simulink model "classd_revb"  (R2024b)
settings: Solver=ode23tb  StartTime=0.0  StopTime=Timespan  MaxStep=classd_maxstep  RelTol=1e-4
InitFcn:
  | p2s_dir = fileparts(get_param(bdroot, 'FileName'));
  | if ~isempty(p2s_dir), addpath(p2s_dir); end
  | clear p2s_dir
  | classd_params;
values from neighbouring files (symbols this model uses):
  Driveshock_freq = 1/(Driveshock_pulse_width*1.25)    (= 72.7272727273)    [classd_params.m]
  Pcd = struct()    [classd_params.m]
  PWMfs = 1/PWMperiod    (= 33333.3333333)    [classd_params.m]
  PWMoffset = PWMperiod/3    (= 1e-05)    [classd_params.m]
  set_current = 450    [classd_params.m]
  shockinterval = 24    [classd_params.m]
  sweep_fEnd = 10000    [classd_params.m]
  sweep_fStart = 4    [classd_params.m]
  tdead = 500e-9    (= 5e-07)    [classd_params.m]
undefined symbols (not defined in the file or in its folder): classd_y0, ipid, vfb
libraries: slpidlib x4
Description:
  | Ideal-switch translation of Class D Rev B.plecs (see README.md)
settings Model: Creator=Jonathan  LastModifiedBy=Jonathan
settings SolverCC: ZeroCrossAlgorithm=Adaptive
settings DebuggingCC: MaxConsecutiveZCsMsg=none

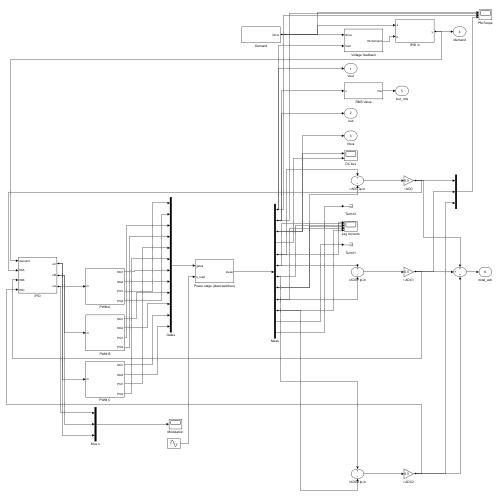
[thumbnail: Simulink's stored preview of the top-level diagram]
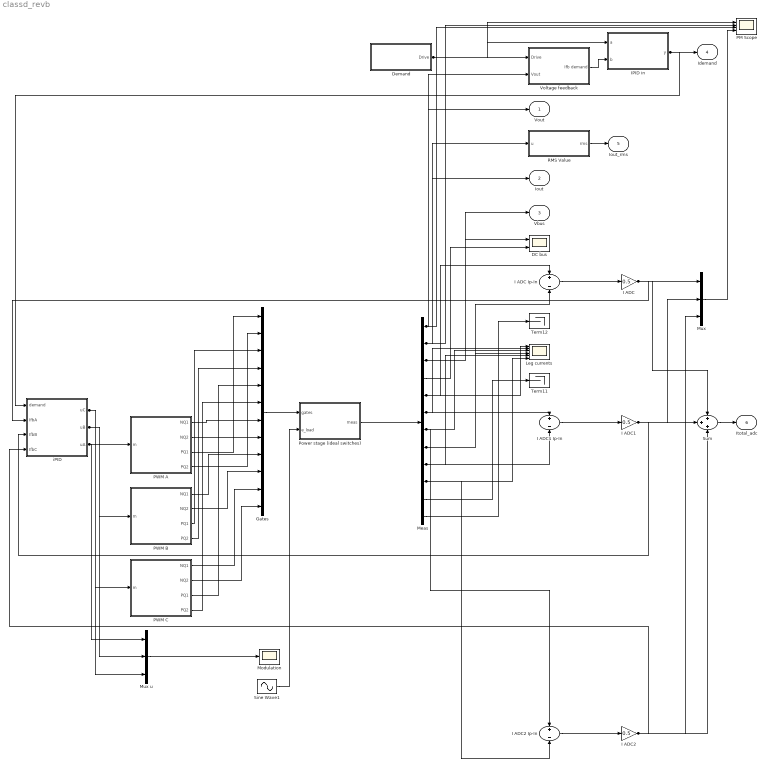
== system classd_revb ==
  DC bus : Scope  NumInputPorts=2
  Demand : Subsystem
  Gates : Mux  Inputs=12
  I ADC : Gain  Gain=0.5
  I ADC Ip-In : Sum  Inputs=+-
  I ADC1 : Gain  Gain=0.5
  I ADC1 Ip-In : Sum  Inputs=+-
  I ADC2 : Gain  Gain=0.5
  I ADC2 Ip-In : Sum  Inputs=+-
  IPID in : Subsystem
  Leg currents : Scope  NumInputPorts=6
  Meas : Demux  Outputs=12
  Modulation : Scope
  Mux : Mux  Inputs=3
  Mux u : Mux  Inputs=3
  PM Scope : Scope  NumInputPorts=4
  PWM A : Subsystem
  PWM B : Subsystem
  PWM C : Subsystem
  Power stage (ideal switches) : Subsystem
  RMS Value : Subsystem
  Sine Wave1 : Sin  Amplitude=10  Frequency=2*pi*20  SampleTime=0
  Sum : Sum  Inputs=+++
  Term11 : Terminator
  Term12 : Terminator
  Voltage feedback : Subsystem
  iPID : Subsystem
  Vout : Outport
  Iout : Outport  Port=2
  Vbus : Outport  Port=3
  Idemand : Outport  Port=4
  Iout_rms : Outport  Port=5
  Itotal_adc : Outport  Port=6
  wires:
  PWM B/4(PQ2) -> Gates/4
  iPID/1(uC) -> PWM C/1(m), Mux u/3
  PWM B/1(NQ1) -> Gates/9
  iPID/2(uB) -> PWM B/1(m), Mux u/2
  iPID/3(uA) -> PWM A/1(m), Mux u/1
  Mux/1 -> PM Scope/4
  PWM A/1(NQ1) -> Gates/7
  PWM A/2(NQ2) -> Gates/8
  PWM A/3(PQ1) -> Gates/1
  PWM A/4(PQ2) -> Gates/2
  PWM B/2(NQ2) -> Gates/10
  PWM B/3(PQ1) -> Gates/3
  Meas/6 -> I ADC1 Ip-In/1, Leg currents/2
  Meas/5 -> Leg currents/1, I ADC Ip-In/1
  PWM C/1(NQ1) -> Gates/11
  PWM C/2(NQ2) -> Gates/12
  Sum/1 -> Itotal_adc/1
  PWM C/4(PQ2) -> Gates/6
  PWM C/3(PQ1) -> Gates/5
  Mux u/1 -> Modulation/1
  Gates/1 -> Power stage (ideal switches)/1(gates)
  Sine Wave1/1 -> Power stage (ideal switches)/2(e_load)
  I ADC1 Ip-In/1 -> I ADC1/1
  Power stage (ideal switches)/1(meas) -> Meas/1
  Demand/1(Drive) -> IPID in/1(a), PM Scope/1, Voltage feedback/1(Drive)
  Meas/2 -> PM Scope/2, RMS Value/1(u), Iout/1
  Meas/1 -> PM Scope/3, Voltage feedback/2(Vout), Vout/1
  Meas/4 -> DC bus/2
  Meas/3 -> DC bus/1, Vbus/1
  Meas/8 -> I ADC Ip-In/2, Leg currents/4
  Meas/7 -> I ADC2 Ip-In/1, Leg currents/3
  Meas/10 -> I ADC2 Ip-In/2, Leg currents/6
  Meas/9 -> I ADC1 Ip-In/2, Leg currents/5
  Meas/12 -> Term12/1
  Meas/11 -> Term11/1
  IPID in/1(y) -> iPID/1(demand), Idemand/1
  Voltage feedback/1(Ifb demand) -> IPID in/2(b)
  RMS Value/1(rms) -> Iout_rms/1
  I ADC Ip-In/1 -> I ADC/1
  I ADC2 Ip-In/1 -> I ADC2/1
  I ADC/1 -> iPID/2(IfbA), Mux/1, Sum/1
  I ADC1/1 -> iPID/3(IfbB), Mux/2, Sum/2
  I ADC2/1 -> iPID/4(IfbC), Sum/3, Mux/3

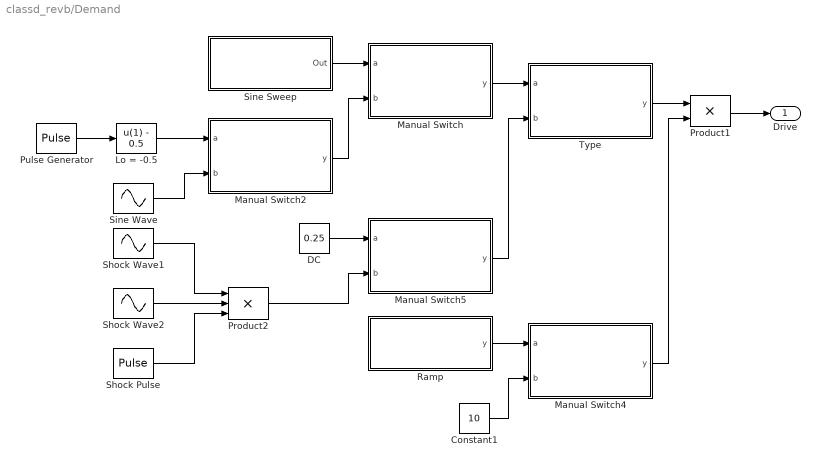
== system classd_revb/Demand ==
  Constant1 : Constant  Value=10
  DC : Constant  Value=0.25
  Lo = -0.5 : Fcn  Expr=u(1) - 0.5
  Manual Switch : Subsystem
  Manual Switch2 : Subsystem
  Manual Switch4 : Subsystem
  Manual Switch5 : Subsystem
  Product1 : Product  Inputs=**
  Product2 : Product  Inputs=***
  Pulse Generator : DiscretePulseGenerator  PulseType=Time based  Period=9/PWMfs  PulseWidth=50  PhaseDelay=0.1
  Ramp : Subsystem
  Shock Pulse : DiscretePulseGenerator  PulseType=Time based  Period=1/(shockinterval*Driveshock_freq/(3*10*2.4))  PulseWidth=100*shockinterval*0.05/2.4
  Shock Wave1 : Sin  Amplitude=set_current  Frequency=2*pi*Driveshock_freq  Phase=-pi  SampleTime=0
  Shock Wave2 : Sin  Amplitude=0.5  Bias=0.5  Frequency=2*pi*Driveshock_freq*2/3  Phase=-pi/2  SampleTime=0
  Sine Sweep : Subsystem
  Sine Wave : Sin  Frequency=2*pi*567.2  SampleTime=0
  Type : Subsystem
  Drive : Outport
  wires:
  Pulse Generator/1 -> Lo = -0.5/1
  Sine Wave/1 -> Manual Switch2/2(b)
  Lo = -0.5/1 -> Manual Switch2/1(a)
  Shock Wave1/1 -> Product2/1
  Sine Sweep/1(Out) -> Manual Switch/1(a)
  Shock Wave2/1 -> Product2/2
  Shock Pulse/1 -> Product2/3
  Manual Switch2/1(y) -> Manual Switch/2(b)
  Product1/1 -> Drive/1
  DC/1 -> Manual Switch5/1(a)
  Product2/1 -> Manual Switch5/2(b)
  Manual Switch/1(y) -> Type/1(a)
  Manual Switch5/1(y) -> Type/2(b)
  Ramp/1(y) -> Manual Switch4/1(a)
  Constant1/1 -> Manual Switch4/2(b)
  Type/1(y) -> Product1/1
  Manual Switch4/1(y) -> Product1/2

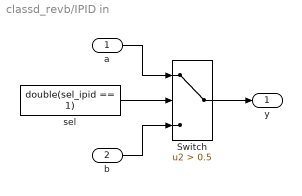
== system classd_revb/IPID in ==
  a : Inport
  b : Inport  Port=2
  Switch : Switch  Criteria=u2 > Threshold  Threshold=0.5  SaturateOnIntegerOverflow=off  InputSameDT=off
  sel : Constant  Value=double(sel_ipid == 1)
  y : Outport
  wires:
  a/1 -> Switch/1
  sel/1 -> Switch/2
  b/1 -> Switch/3
  Switch/1 -> y/1

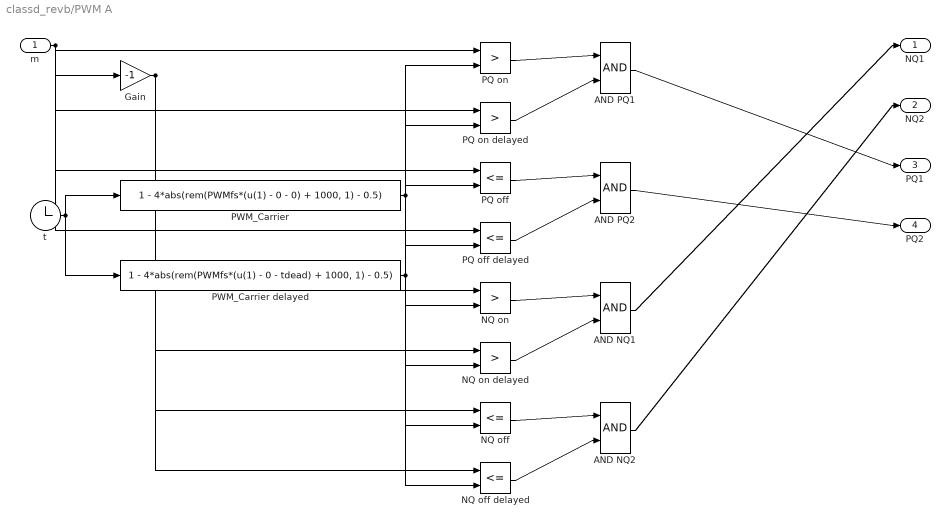
== system classd_revb/PWM A ==
  m : Inport
  AND NQ1 : Logic  AllPortsSameDT=off  OutDataTypeStr=boolean
  AND NQ2 : Logic  AllPortsSameDT=off  OutDataTypeStr=boolean
  AND PQ1 : Logic  AllPortsSameDT=off  OutDataTypeStr=boolean
  AND PQ2 : Logic  AllPortsSameDT=off  OutDataTypeStr=boolean
  Gain : Gain  Gain=-1
  NQ off : RelationalOperator  Operator=<=  OutDataTypeStr=boolean  RndMeth=Simplest  InputSameDT=off
  NQ off delayed : RelationalOperator  Operator=<=  OutDataTypeStr=boolean  RndMeth=Simplest  InputSameDT=off
  NQ on : RelationalOperator  Operator=>  OutDataTypeStr=boolean  RndMeth=Simplest  InputSameDT=off
  NQ on delayed : RelationalOperator  Operator=>  OutDataTypeStr=boolean  RndMeth=Simplest  InputSameDT=off
  PQ off : RelationalOperator  Operator=<=  OutDataTypeStr=boolean  RndMeth=Simplest  InputSameDT=off
  PQ off delayed : RelationalOperator  Operator=<=  OutDataTypeStr=boolean  RndMeth=Simplest  InputSameDT=off
  PQ on : RelationalOperator  Operator=>  OutDataTypeStr=boolean  RndMeth=Simplest  InputSameDT=off
  PQ on delayed : RelationalOperator  Operator=>  OutDataTypeStr=boolean  RndMeth=Simplest  InputSameDT=off
  PWM_Carrier : Fcn  Expr=1 - 4*abs(rem(PWMfs*(u(1) - 0 - 0) + 1000, 1) - 0.5)
  PWM_Carrier delayed : Fcn  Expr=1 - 4*abs(rem(PWMfs*(u(1) - 0 - tdead) + 1000, 1) - 0.5)
  t : Clock
  NQ1 : Outport
  NQ2 : Outport  Port=2
  PQ1 : Outport  Port=3
  PQ2 : Outport  Port=4
  wires:
  t/1 -> PWM_Carrier/1, PWM_Carrier delayed/1
  m/1 -> Gain/1, PQ on/1, PQ on delayed/1, PQ off/1, PQ off delayed/1
  PWM_Carrier/1 -> PQ on/2, PQ off/2, NQ on/2, NQ off/2
  PWM_Carrier delayed/1 -> PQ on delayed/2, PQ off delayed/2, NQ on delayed/2, NQ off delayed/2
  PQ on/1 -> AND PQ1/1
  PQ on delayed/1 -> AND PQ1/2
  PQ off/1 -> AND PQ2/1
  PQ off delayed/1 -> AND PQ2/2
  AND PQ1/1 -> PQ1/1
  AND PQ2/1 -> PQ2/1
  Gain/1 -> NQ on/1, NQ on delayed/1, NQ off/1, NQ off delayed/1
  NQ on/1 -> AND NQ1/1
  NQ on delayed/1 -> AND NQ1/2
  NQ off/1 -> AND NQ2/1
  NQ off delayed/1 -> AND NQ2/2
  AND NQ1/1 -> NQ1/1
  AND NQ2/1 -> NQ2/1

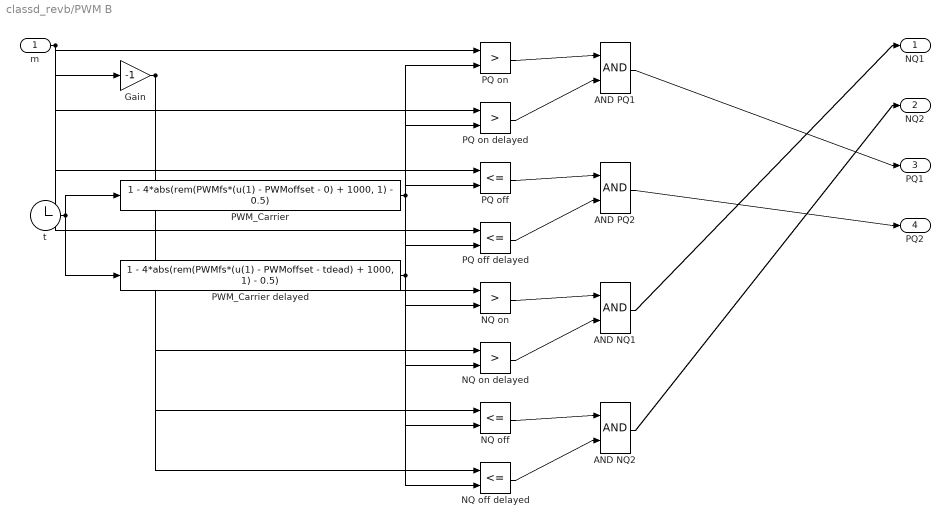
== system classd_revb/PWM B ==
  m : Inport
  AND NQ1 : Logic  AllPortsSameDT=off  OutDataTypeStr=boolean
  AND NQ2 : Logic  AllPortsSameDT=off  OutDataTypeStr=boolean
  AND PQ1 : Logic  AllPortsSameDT=off  OutDataTypeStr=boolean
  AND PQ2 : Logic  AllPortsSameDT=off  OutDataTypeStr=boolean
  Gain : Gain  Gain=-1
  NQ off : RelationalOperator  Operator=<=  OutDataTypeStr=boolean  RndMeth=Simplest  InputSameDT=off
  NQ off delayed : RelationalOperator  Operator=<=  OutDataTypeStr=boolean  RndMeth=Simplest  InputSameDT=off
  NQ on : RelationalOperator  Operator=>  OutDataTypeStr=boolean  RndMeth=Simplest  InputSameDT=off
  NQ on delayed : RelationalOperator  Operator=>  OutDataTypeStr=boolean  RndMeth=Simplest  InputSameDT=off
  PQ off : RelationalOperator  Operator=<=  OutDataTypeStr=boolean  RndMeth=Simplest  InputSameDT=off
  PQ off delayed : RelationalOperator  Operator=<=  OutDataTypeStr=boolean  RndMeth=Simplest  InputSameDT=off
  PQ on : RelationalOperator  Operator=>  OutDataTypeStr=boolean  RndMeth=Simplest  InputSameDT=off
  PQ on delayed : RelationalOperator  Operator=>  OutDataTypeStr=boolean  RndMeth=Simplest  InputSameDT=off
  PWM_Carrier : Fcn  Expr=1 - 4*abs(rem(PWMfs*(u(1) - PWMoffset - 0) + 1000, 1) - 0.5)
  PWM_Carrier delayed : Fcn  Expr=1 - 4*abs(rem(PWMfs*(u(1) - PWMoffset - tdead) + 1000, 1) - 0.5)
  t : Clock
  NQ1 : Outport
  NQ2 : Outport  Port=2
  PQ1 : Outport  Port=3
  PQ2 : Outport  Port=4
  wires:
  t/1 -> PWM_Carrier/1, PWM_Carrier delayed/1
  m/1 -> Gain/1, PQ on/1, PQ on delayed/1, PQ off/1, PQ off delayed/1
  PWM_Carrier/1 -> PQ on/2, PQ off/2, NQ on/2, NQ off/2
  PWM_Carrier delayed/1 -> PQ on delayed/2, PQ off delayed/2, NQ on delayed/2, NQ off delayed/2
  PQ on/1 -> AND PQ1/1
  PQ on delayed/1 -> AND PQ1/2
  PQ off/1 -> AND PQ2/1
  PQ off delayed/1 -> AND PQ2/2
  AND PQ1/1 -> PQ1/1
  AND PQ2/1 -> PQ2/1
  Gain/1 -> NQ on/1, NQ on delayed/1, NQ off/1, NQ off delayed/1
  NQ on/1 -> AND NQ1/1
  NQ on delayed/1 -> AND NQ1/2
  NQ off/1 -> AND NQ2/1
  NQ off delayed/1 -> AND NQ2/2
  AND NQ1/1 -> NQ1/1
  AND NQ2/1 -> NQ2/1

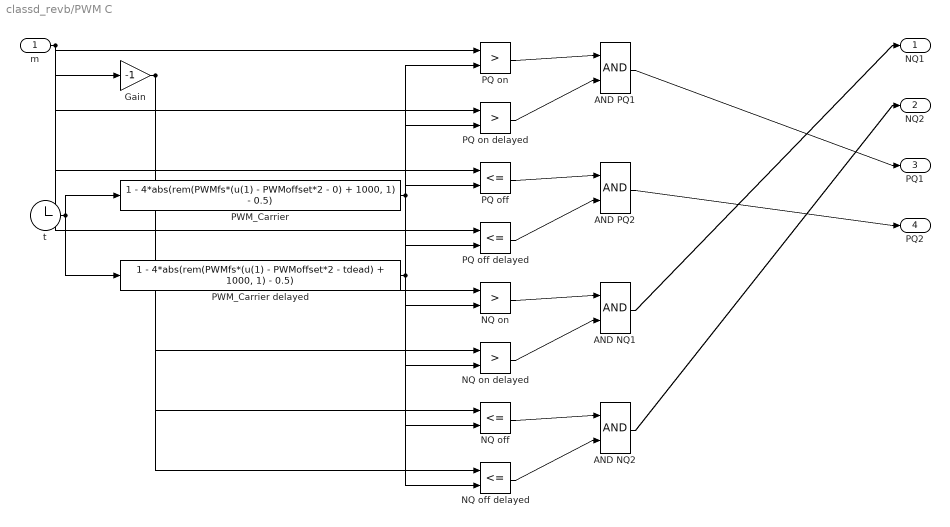
== system classd_revb/PWM C ==
  m : Inport
  AND NQ1 : Logic  AllPortsSameDT=off  OutDataTypeStr=boolean
  AND NQ2 : Logic  AllPortsSameDT=off  OutDataTypeStr=boolean
  AND PQ1 : Logic  AllPortsSameDT=off  OutDataTypeStr=boolean
  AND PQ2 : Logic  AllPortsSameDT=off  OutDataTypeStr=boolean
  Gain : Gain  Gain=-1
  NQ off : RelationalOperator  Operator=<=  OutDataTypeStr=boolean  RndMeth=Simplest  InputSameDT=off
  NQ off delayed : RelationalOperator  Operator=<=  OutDataTypeStr=boolean  RndMeth=Simplest  InputSameDT=off
  NQ on : RelationalOperator  Operator=>  OutDataTypeStr=boolean  RndMeth=Simplest  InputSameDT=off
  NQ on delayed : RelationalOperator  Operator=>  OutDataTypeStr=boolean  RndMeth=Simplest  InputSameDT=off
  PQ off : RelationalOperator  Operator=<=  OutDataTypeStr=boolean  RndMeth=Simplest  InputSameDT=off
  PQ off delayed : RelationalOperator  Operator=<=  OutDataTypeStr=boolean  RndMeth=Simplest  InputSameDT=off
  PQ on : RelationalOperator  Operator=>  OutDataTypeStr=boolean  RndMeth=Simplest  InputSameDT=off
  PQ on delayed : RelationalOperator  Operator=>  OutDataTypeStr=boolean  RndMeth=Simplest  InputSameDT=off
  PWM_Carrier : Fcn  Expr=1 - 4*abs(rem(PWMfs*(u(1) - PWMoffset*2 - 0) + 1000, 1) - 0.5)
  PWM_Carrier delayed : Fcn  Expr=1 - 4*abs(rem(PWMfs*(u(1) - PWMoffset*2 - tdead) + 1000, 1) - 0.5)
  t : Clock
  NQ1 : Outport
  NQ2 : Outport  Port=2
  PQ1 : Outport  Port=3
  PQ2 : Outport  Port=4
  wires:
  t/1 -> PWM_Carrier/1, PWM_Carrier delayed/1
  m/1 -> Gain/1, PQ on/1, PQ on delayed/1, PQ off/1, PQ off delayed/1
  PWM_Carrier/1 -> PQ on/2, PQ off/2, NQ on/2, NQ off/2
  PWM_Carrier delayed/1 -> PQ on delayed/2, PQ off delayed/2, NQ on delayed/2, NQ off delayed/2
  PQ on/1 -> AND PQ1/1
  PQ on delayed/1 -> AND PQ1/2
  PQ off/1 -> AND PQ2/1
  PQ off delayed/1 -> AND PQ2/2
  AND PQ1/1 -> PQ1/1
  AND PQ2/1 -> PQ2/1
  Gain/1 -> NQ on/1, NQ on delayed/1, NQ off/1, NQ off delayed/1
  NQ on/1 -> AND NQ1/1
  NQ on delayed/1 -> AND NQ1/2
  NQ off/1 -> AND NQ2/1
  NQ off delayed/1 -> AND NQ2/2
  AND NQ1/1 -> NQ1/1
  AND NQ2/1 -> NQ2/1

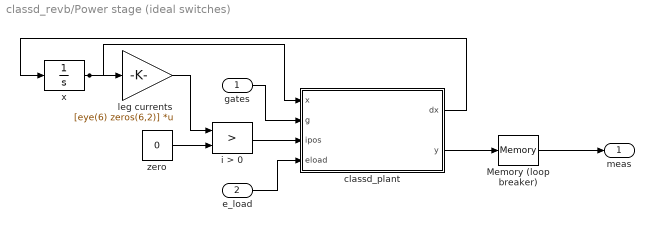
== system classd_revb/Power stage (ideal switches) ==
  gates : Inport
  e_load : Inport  Port=2
  Memory (loop breaker) : Memory  InitialCondition=classd_y0
  classd_plant : MATLAB Function  TreatAsAtomicUnit=on
  i > 0 : RelationalOperator  Operator=>  OutDataTypeStr=boolean  RndMeth=Simplest  InputSameDT=off
  leg currents : Gain  Gain=[eye(6) zeros(6,2)]  Multiplication=Matrix(K*u)
  x : Integrator  InitialCondition=Pcd.x0
  zero : Constant  Value=0
  meas : Outport
  wires:
  classd_plant/2(y) -> Memory (loop breaker)/1
  x/1 -> classd_plant/1(x), leg currents/1
  leg currents/1 -> i > 0/1
  classd_plant/1(dx) -> x/1
  zero/1 -> i > 0/2
  e_load/1 -> classd_plant/4(eload)
  gates/1 -> classd_plant/2(g)
  i > 0/1 -> classd_plant/3(ipos)
  Memory (loop breaker)/1 -> meas/1

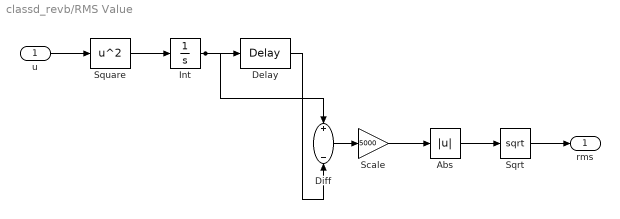
== system classd_revb/RMS Value ==
  u : Inport
  Abs : Abs  SaturateOnIntegerOverflow=off
  Delay : TransportDelay  DelayTime=1/(5000)  BufferSize=131072
  Diff : Sum  Inputs=+-
  Int : Integrator
  Scale : Gain  Gain=5000
  Sqrt : Sqrt
  Square : Math  Operator=square
  rms : Outport
  wires:
  Diff/1 -> Scale/1
  u/1 -> Square/1
  Square/1 -> Int/1
  Delay/1 -> Diff/2
  Int/1 -> Diff/1, Delay/1
  Scale/1 -> Abs/1
  Abs/1 -> Sqrt/1
  Sqrt/1 -> rms/1

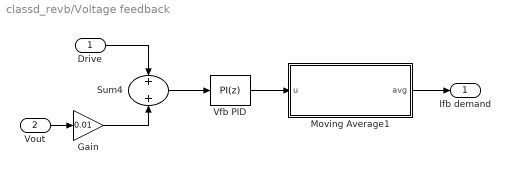
== system classd_revb/Voltage feedback ==
  Drive : Inport
  Vout : Inport  Port=2
  Gain : Gain  Gain=0.01
  Moving Average1 : Subsystem
  Sum4 : Sum
  Vfb PID : slpidlib/PID Controller  Controller=PI  Form=Parallel  TimeDomain=Discrete-time  UseExternalTs=off  SampleTime=vfb.Ts  IntegratorMethod=Forward Euler  FilterMethod=Forward Euler  ControllerParametersSource=internal  P=vfb.kp  I=vfb.ki  UseKiTs=off  D=0  UseExternalDerivativeSource=off  N=100  UseFilter=on  TunerSelectOption=Transfer Function Based (PID Tuner App)  InitialConditionSource=internal  InitialConditionForIntegrator=0  InitialConditionForFilter=0  DifferentiatorICPrevScaledInput=0  ExternalReset=none  TrackingMode=off  Kt=1  LimitOutput=on  SatLimitsSource=internal  UpperSaturationLimit=vfb.up  LowerSaturationLimit=vfb.lo  LinearizeAsGain=off  AntiWindupMode=clamping  Kb=1  LimitIntegrator=off  UpperIntegratorSaturationLimit=inf  LowerIntegratorSaturationLimit=-inf  POutMin=[]  POutMax=[]  IOutMin=[]  IOutMax=[]  DOutMin=[]  DOutMax=[]  NOutMin=[]  NOutMax=[]  SumOutMin=[]  SumOutMax=[]  SaturationOutMin=[]  SaturationOutMax=[]  PParamMin=[]  PParamMax=[]  IParamMin=[]  IParamMax=[]  DParamMin=[]  DParamMax=[]  NParamMin=[]  NParamMax=[]  KbParamMin=[]  KbParamMax=[]  KtParamMin=[]  KtParamMax=[]  KbOutMin=[]  KbOutMax=[]  KtOutMin=[]  KtOutMax=[]  IntegratorOutMin=[]  IntegratorOutMax=[]  FilterOutMin=[]  FilterOutMax=[]  SumI1OutMin=[]  SumI1OutMax=[]  SumI2OutMin=[]  SumI2OutMax=[]  SumI3OutMin=[]  SumI3OutMax=[]  SumI4OutMin=[]  SumI4OutMax=[]  SumDOutMin=[]  SumDOutMax=[]  DifferentiatorOutMin=[]  DifferentiatorOutMax=[]  FilterDiffOutCoefMin=[]  FilterDiffOutCoefMax=[]  ReciprocalOutMin=[]  ReciprocalOutMax=[]  SumDenOutMin=[]  SumDenOutMax=[]  SumNumOutMin=[]  SumNumOutMax=[]  DivideOutMin=[]  DivideOutMax=[]  UdiffTsProdOutMin=[]  UdiffTsProdOutMax=[]  NTsProdOutMin=[]  NTsProdOutMax=[]  UintegralTsProdOutMin=[]  UintegralTsProdOutMax=[]  UngainTsProdOutMin=[]  UngainTsProdOutMax=[]  ClampingZeroOutDataTypeStr=Inherit: Inherit via back propagation  ClampingZeroOutMin=[]  ClampingZeroOutMax=[]  FilterDenConstantOutDataTypeStr=Inherit: Inherit via back propagation  FilterDenConstantOutMin=[]  FilterDenConstantOutMax=[]  PCopyOutDataTypeStr=Inherit: Inherit via back propagation  PCopyOutMin=[]  PCopyOutMax=[]  NCopyOutDataTypeStr=Inherit: Inherit via back propagation  NCopyOutMin=[]  NCopyOutMax=[]  IntegratorContinuousStateAttributes=''  IntegratorStateMustResolveToSignalObject=off  IntegratorRTWStateStorageClass=Auto  FilterContinuousStateAttributes=''  FilterStateMustResolveToSignalObject=off  FilterRTWStateStorageClass=Auto  ParallelPVariant=InternalParameters  IdealPVariant=Disabled  IVariant=InternalParameters  DVariant=Disabled  IntegratorVariant=Discrete  SatVariant=Enabled  AWVariant=DiscClampingParallel  PCopyVariant=Disabled  TRVariant=Disabled  FdbkBlocksVariant=Forward  IdealPFdbkVariant=Disabled  SatFdbkVariant=Disabled  DerivativeFilterVariant=Disabled  NVariant=Disabled  NCopyVariant=Disabled_SignalSpec  FilterICVariant=Disabled  IntegratorICVariant=InternalICs  ExternalResetVariant=Disabled  TRSumVariant=Passthrough  SumFdbkVariant=Disabled  SumVariant=Sum_PI  TsampFilterVariant=InternalTs  TsampNgainVariant=Passthrough  TsampIntegralVariant=Disabled_SignalSpec  ExternalSaturationOutDataTypeStr=Inherit: Same as second input  DerivativeSourceVariant=Disabled  PreIntVariant=InternalPreInt
      settings: LibrarySourceBlock=simulink/Discrete/Discrete PID Controller
  Ifb demand : Outport
  wires:
  Vout/1 -> Gain/1
  Moving Average1/1(avg) -> Ifb demand/1
  Drive/1 -> Sum4/1
  Gain/1 -> Sum4/2
  Sum4/1 -> Vfb PID/1
  Vfb PID/1 -> Moving Average1/1(u)

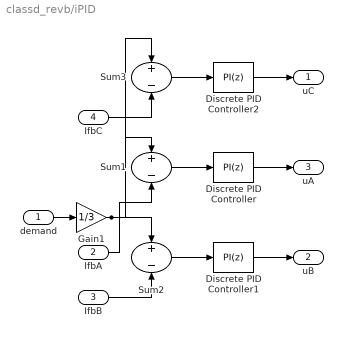
== system classd_revb/iPID ==
  demand : Inport
  IfbA : Inport  Port=2
  IfbB : Inport  Port=3
  IfbC : Inport  Port=4
  Discrete PID Controller : slpidlib/PID Controller  Controller=PI  Form=Parallel  TimeDomain=Discrete-time  UseExternalTs=off  SampleTime=ipid.Ts  IntegratorMethod=Forward Euler  FilterMethod=Forward Euler  ControllerParametersSource=internal  P=ipid.kp  I=ipid.ki  UseKiTs=off  D=0  UseExternalDerivativeSource=off  N=100  UseFilter=on  TunerSelectOption=Transfer Function Based (PID Tuner App)  InitialConditionSource=internal  InitialConditionForIntegrator=0  InitialConditionForFilter=0  DifferentiatorICPrevScaledInput=0  ExternalReset=none  TrackingMode=off  Kt=1  LimitOutput=on  SatLimitsSource=internal  UpperSaturationLimit=ipid.up  LowerSaturationLimit=ipid.lo  LinearizeAsGain=off  AntiWindupMode=back-calculation  Kb=ipid.kbc  LimitIntegrator=off  UpperIntegratorSaturationLimit=inf  LowerIntegratorSaturationLimit=-inf  POutMin=[]  POutMax=[]  IOutMin=[]  IOutMax=[]  DOutMin=[]  DOutMax=[]  NOutMin=[]  NOutMax=[]  SumOutMin=[]  SumOutMax=[]  SaturationOutMin=[]  SaturationOutMax=[]  PParamMin=[]  PParamMax=[]  IParamMin=[]  IParamMax=[]  DParamMin=[]  DParamMax=[]  NParamMin=[]  NParamMax=[]  KbParamMin=[]  KbParamMax=[]  KtParamMin=[]  KtParamMax=[]  KbOutMin=[]  KbOutMax=[]  KtOutMin=[]  KtOutMax=[]  IntegratorOutMin=[]  IntegratorOutMax=[]  FilterOutMin=[]  FilterOutMax=[]  SumI1OutMin=[]  SumI1OutMax=[]  SumI2OutMin=[]  SumI2OutMax=[]  SumI3OutMin=[]  SumI3OutMax=[]  SumI4OutMin=[]  SumI4OutMax=[]  SumDOutMin=[]  SumDOutMax=[]  DifferentiatorOutMin=[]  DifferentiatorOutMax=[]  FilterDiffOutCoefMin=[]  FilterDiffOutCoefMax=[]  ReciprocalOutMin=[]  ReciprocalOutMax=[]  SumDenOutMin=[]  SumDenOutMax=[]  SumNumOutMin=[]  SumNumOutMax=[]  DivideOutMin=[]  DivideOutMax=[]  UdiffTsProdOutMin=[]  UdiffTsProdOutMax=[]  NTsProdOutMin=[]  NTsProdOutMax=[]  UintegralTsProdOutMin=[]  UintegralTsProdOutMax=[]  UngainTsProdOutMin=[]  UngainTsProdOutMax=[]  ClampingZeroOutDataTypeStr=Inherit: Inherit via back propagation  ClampingZeroOutMin=[]  ClampingZeroOutMax=[]  FilterDenConstantOutDataTypeStr=Inherit: Inherit via back propagation  FilterDenConstantOutMin=[]  FilterDenConstantOutMax=[]  PCopyOutDataTypeStr=Inherit: Inherit via back propagation  PCopyOutMin=[]  PCopyOutMax=[]  NCopyOutDataTypeStr=Inherit: Inherit via back propagation  NCopyOutMin=[]  NCopyOutMax=[]  IntegratorContinuousStateAttributes=''  IntegratorStateMustResolveToSignalObject=off  IntegratorRTWStateStorageClass=Auto  FilterContinuousStateAttributes=''  FilterStateMustResolveToSignalObject=off  FilterRTWStateStorageClass=Auto  ParallelPVariant=InternalParameters  IdealPVariant=Disabled  IVariant=InternalParameters  DVariant=Disabled  IntegratorVariant=Discrete  SatVariant=Enabled  AWVariant=BackCalculation  PCopyVariant=Disabled  TRVariant=Disabled  FdbkBlocksVariant=Forward  IdealPFdbkVariant=Disabled  SatFdbkVariant=Disabled  DerivativeFilterVariant=Disabled  NVariant=Disabled  NCopyVariant=Disabled_SignalSpec  FilterICVariant=Disabled  IntegratorICVariant=InternalICs  ExternalResetVariant=Disabled  TRSumVariant=Passthrough  SumFdbkVariant=Disabled  SumVariant=Sum_PI  TsampFilterVariant=InternalTs  TsampNgainVariant=Passthrough  TsampIntegralVariant=Disabled_SignalSpec  ExternalSaturationOutDataTypeStr=Inherit: Same as second input  DerivativeSourceVariant=Disabled  PreIntVariant=InternalPreInt
      settings: LibrarySourceBlock=simulink/Discrete/Discrete PID Controller
  Discrete PID Controller1 : slpidlib/PID Controller  Controller=PI  Form=Parallel  TimeDomain=Discrete-time  UseExternalTs=off  SampleTime=ipid.Ts  IntegratorMethod=Forward Euler  FilterMethod=Forward Euler  ControllerParametersSource=internal  P=ipid.kp  I=ipid.ki  UseKiTs=off  D=0  UseExternalDerivativeSource=off  N=100  UseFilter=on  TunerSelectOption=Transfer Function Based (PID Tuner App)  InitialConditionSource=internal  InitialConditionForIntegrator=0  InitialConditionForFilter=0  DifferentiatorICPrevScaledInput=0  ExternalReset=none  TrackingMode=off  Kt=1  LimitOutput=on  SatLimitsSource=internal  UpperSaturationLimit=ipid.up  LowerSaturationLimit=ipid.lo  LinearizeAsGain=off  AntiWindupMode=back-calculation  Kb=ipid.kbc  LimitIntegrator=off  UpperIntegratorSaturationLimit=inf  LowerIntegratorSaturationLimit=-inf  POutMin=[]  POutMax=[]  IOutMin=[]  IOutMax=[]  DOutMin=[]  DOutMax=[]  NOutMin=[]  NOutMax=[]  SumOutMin=[]  SumOutMax=[]  SaturationOutMin=[]  SaturationOutMax=[]  PParamMin=[]  PParamMax=[]  IParamMin=[]  IParamMax=[]  DParamMin=[]  DParamMax=[]  NParamMin=[]  NParamMax=[]  KbParamMin=[]  KbParamMax=[]  KtParamMin=[]  KtParamMax=[]  KbOutMin=[]  KbOutMax=[]  KtOutMin=[]  KtOutMax=[]  IntegratorOutMin=[]  IntegratorOutMax=[]  FilterOutMin=[]  FilterOutMax=[]  SumI1OutMin=[]  SumI1OutMax=[]  SumI2OutMin=[]  SumI2OutMax=[]  SumI3OutMin=[]  SumI3OutMax=[]  SumI4OutMin=[]  SumI4OutMax=[]  SumDOutMin=[]  SumDOutMax=[]  DifferentiatorOutMin=[]  DifferentiatorOutMax=[]  FilterDiffOutCoefMin=[]  FilterDiffOutCoefMax=[]  ReciprocalOutMin=[]  ReciprocalOutMax=[]  SumDenOutMin=[]  SumDenOutMax=[]  SumNumOutMin=[]  SumNumOutMax=[]  DivideOutMin=[]  DivideOutMax=[]  UdiffTsProdOutMin=[]  UdiffTsProdOutMax=[]  NTsProdOutMin=[]  NTsProdOutMax=[]  UintegralTsProdOutMin=[]  UintegralTsProdOutMax=[]  UngainTsProdOutMin=[]  UngainTsProdOutMax=[]  ClampingZeroOutDataTypeStr=Inherit: Inherit via back propagation  ClampingZeroOutMin=[]  ClampingZeroOutMax=[]  FilterDenConstantOutDataTypeStr=Inherit: Inherit via back propagation  FilterDenConstantOutMin=[]  FilterDenConstantOutMax=[]  PCopyOutDataTypeStr=Inherit: Inherit via back propagation  PCopyOutMin=[]  PCopyOutMax=[]  NCopyOutDataTypeStr=Inherit: Inherit via back propagation  NCopyOutMin=[]  NCopyOutMax=[]  IntegratorContinuousStateAttributes=''  IntegratorStateMustResolveToSignalObject=off  IntegratorRTWStateStorageClass=Auto  FilterContinuousStateAttributes=''  FilterStateMustResolveToSignalObject=off  FilterRTWStateStorageClass=Auto  ParallelPVariant=InternalParameters  IdealPVariant=Disabled  IVariant=InternalParameters  DVariant=Disabled  IntegratorVariant=Discrete  SatVariant=Enabled  AWVariant=BackCalculation  PCopyVariant=Disabled  TRVariant=Disabled  FdbkBlocksVariant=Forward  IdealPFdbkVariant=Disabled  SatFdbkVariant=Disabled  DerivativeFilterVariant=Disabled  NVariant=Disabled  NCopyVariant=Disabled_SignalSpec  FilterICVariant=Disabled  IntegratorICVariant=InternalICs  ExternalResetVariant=Disabled  TRSumVariant=Passthrough  SumFdbkVariant=Disabled  SumVariant=Sum_PI  TsampFilterVariant=InternalTs  TsampNgainVariant=Passthrough  TsampIntegralVariant=Disabled_SignalSpec  ExternalSaturationOutDataTypeStr=Inherit: Same as second input  DerivativeSourceVariant=Disabled  PreIntVariant=InternalPreInt
      settings: LibrarySourceBlock=simulink/Discrete/Discrete PID Controller
  Discrete PID Controller2 : slpidlib/PID Controller  Controller=PI  Form=Parallel  TimeDomain=Discrete-time  UseExternalTs=off  SampleTime=ipid.Ts  IntegratorMethod=Forward Euler  FilterMethod=Forward Euler  ControllerParametersSource=internal  P=ipid.kp  I=ipid.ki  UseKiTs=off  D=0  UseExternalDerivativeSource=off  N=100  UseFilter=on  TunerSelectOption=Transfer Function Based (PID Tuner App)  InitialConditionSource=internal  InitialConditionForIntegrator=0  InitialConditionForFilter=0  DifferentiatorICPrevScaledInput=0  ExternalReset=none  TrackingMode=off  Kt=1  LimitOutput=on  SatLimitsSource=internal  UpperSaturationLimit=ipid.up  LowerSaturationLimit=ipid.lo  LinearizeAsGain=off  AntiWindupMode=back-calculation  Kb=ipid.kbc  LimitIntegrator=off  UpperIntegratorSaturationLimit=inf  LowerIntegratorSaturationLimit=-inf  POutMin=[]  POutMax=[]  IOutMin=[]  IOutMax=[]  DOutMin=[]  DOutMax=[]  NOutMin=[]  NOutMax=[]  SumOutMin=[]  SumOutMax=[]  SaturationOutMin=[]  SaturationOutMax=[]  PParamMin=[]  PParamMax=[]  IParamMin=[]  IParamMax=[]  DParamMin=[]  DParamMax=[]  NParamMin=[]  NParamMax=[]  KbParamMin=[]  KbParamMax=[]  KtParamMin=[]  KtParamMax=[]  KbOutMin=[]  KbOutMax=[]  KtOutMin=[]  KtOutMax=[]  IntegratorOutMin=[]  IntegratorOutMax=[]  FilterOutMin=[]  FilterOutMax=[]  SumI1OutMin=[]  SumI1OutMax=[]  SumI2OutMin=[]  SumI2OutMax=[]  SumI3OutMin=[]  SumI3OutMax=[]  SumI4OutMin=[]  SumI4OutMax=[]  SumDOutMin=[]  SumDOutMax=[]  DifferentiatorOutMin=[]  DifferentiatorOutMax=[]  FilterDiffOutCoefMin=[]  FilterDiffOutCoefMax=[]  ReciprocalOutMin=[]  ReciprocalOutMax=[]  SumDenOutMin=[]  SumDenOutMax=[]  SumNumOutMin=[]  SumNumOutMax=[]  DivideOutMin=[]  DivideOutMax=[]  UdiffTsProdOutMin=[]  UdiffTsProdOutMax=[]  NTsProdOutMin=[]  NTsProdOutMax=[]  UintegralTsProdOutMin=[]  UintegralTsProdOutMax=[]  UngainTsProdOutMin=[]  UngainTsProdOutMax=[]  ClampingZeroOutDataTypeStr=Inherit: Inherit via back propagation  ClampingZeroOutMin=[]  ClampingZeroOutMax=[]  FilterDenConstantOutDataTypeStr=Inherit: Inherit via back propagation  FilterDenConstantOutMin=[]  FilterDenConstantOutMax=[]  PCopyOutDataTypeStr=Inherit: Inherit via back propagation  PCopyOutMin=[]  PCopyOutMax=[]  NCopyOutDataTypeStr=Inherit: Inherit via back propagation  NCopyOutMin=[]  NCopyOutMax=[]  IntegratorContinuousStateAttributes=''  IntegratorStateMustResolveToSignalObject=off  IntegratorRTWStateStorageClass=Auto  FilterContinuousStateAttributes=''  FilterStateMustResolveToSignalObject=off  FilterRTWStateStorageClass=Auto  ParallelPVariant=InternalParameters  IdealPVariant=Disabled  IVariant=InternalParameters  DVariant=Disabled  IntegratorVariant=Discrete  SatVariant=Enabled  AWVariant=BackCalculation  PCopyVariant=Disabled  TRVariant=Disabled  FdbkBlocksVariant=Forward  IdealPFdbkVariant=Disabled  SatFdbkVariant=Disabled  DerivativeFilterVariant=Disabled  NVariant=Disabled  NCopyVariant=Disabled_SignalSpec  FilterICVariant=Disabled  IntegratorICVariant=InternalICs  ExternalResetVariant=Disabled  TRSumVariant=Passthrough  SumFdbkVariant=Disabled  SumVariant=Sum_PI  TsampFilterVariant=InternalTs  TsampNgainVariant=Passthrough  TsampIntegralVariant=Disabled_SignalSpec  ExternalSaturationOutDataTypeStr=Inherit: Same as second input  DerivativeSourceVariant=Disabled  PreIntVariant=InternalPreInt
      settings: LibrarySourceBlock=simulink/Discrete/Discrete PID Controller
  Gain1 : Gain  Gain=1/3
  Sum1 : Sum  Inputs=+-
  Sum2 : Sum  Inputs=+-
  Sum3 : Sum  Inputs=+-
  uC : Outport
  uB : Outport  Port=2
  uA : Outport  Port=3
  wires:
  demand/1 -> Gain1/1
  IfbC/1 -> Sum3/2
  IfbB/1 -> Sum2/2
  Gain1/1 -> Sum1/1, Sum2/1, Sum3/1
  IfbA/1 -> Sum1/2
  Sum1/1 -> Discrete PID Controller/1
  Sum2/1 -> Discrete PID Controller1/1
  Sum3/1 -> Discrete PID Controller2/1
  Discrete PID Controller2/1 -> uC/1
  Discrete PID Controller/1 -> uA/1
  Discrete PID Controller1/1 -> uB/1

== system classd_revb/Demand/Manual Switch ==
  a : Inport
  b : Inport  Port=2
  Switch : Switch  Criteria=u2 > Threshold  Threshold=0.5  SaturateOnIntegerOverflow=off  InputSameDT=off
  sel : Constant  Value=double(sel_ms == 1)
  y : Outport
  wires:
  a/1 -> Switch/1
  sel/1 -> Switch/2
  b/1 -> Switch/3
  Switch/1 -> y/1

== system classd_revb/Demand/Manual Switch2 ==
  a : Inport
  b : Inport  Port=2
  Switch : Switch  Criteria=u2 > Threshold  Threshold=0.5  SaturateOnIntegerOverflow=off  InputSameDT=off
  sel : Constant  Value=double(sel_ms2 == 1)
  y : Outport
  wires:
  a/1 -> Switch/1
  sel/1 -> Switch/2
  b/1 -> Switch/3
  Switch/1 -> y/1

== system classd_revb/Demand/Manual Switch4 ==
  a : Inport
  b : Inport  Port=2
  Switch : Switch  Criteria=u2 > Threshold  Threshold=0.5  SaturateOnIntegerOverflow=off  InputSameDT=off
  sel : Constant  Value=double(sel_ms4 == 1)
  y : Outport
  wires:
  a/1 -> Switch/1
  sel/1 -> Switch/2
  b/1 -> Switch/3
  Switch/1 -> y/1

== system classd_revb/Demand/Manual Switch5 ==
  a : Inport
  b : Inport  Port=2
  Switch : Switch  Criteria=u2 > Threshold  Threshold=0.5  SaturateOnIntegerOverflow=off  InputSameDT=off
  sel : Constant  Value=double(sel_ms5 == 1)
  y : Outport
  wires:
  a/1 -> Switch/1
  sel/1 -> Switch/2
  b/1 -> Switch/3
  Switch/1 -> y/1

== system classd_revb/Demand/Ramp ==
  Limit : Saturate  UpperLimit=max(0,120)  LowerLimit=min(0,120)
  Ramp : Fcn  Expr=(0) + (120*(1/Timespan))*(u(1)-(0))*(u(1)>(0))
  t : Clock
  y : Outport
  wires:
  t/1 -> Ramp/1
  Ramp/1 -> Limit/1
  Limit/1 -> y/1

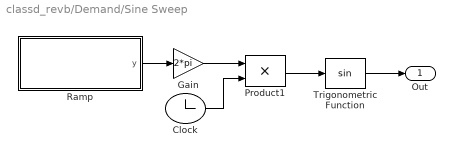
== system classd_revb/Demand/Sine Sweep ==
  Clock : Clock
  Gain : Gain  Gain=2*pi
  Product1 : Product  Inputs=**
  Ramp : Subsystem
  Trigonometric Function : Trigonometry
  Out : Outport
  wires:
  Clock/1 -> Product1/2
  Ramp/1(y) -> Gain/1
  Gain/1 -> Product1/1
  Product1/1 -> Trigonometric Function/1
  Trigonometric Function/1 -> Out/1

== system classd_revb/Demand/Type ==
  a : Inport
  b : Inport  Port=2
  Switch : Switch  Criteria=u2 > Threshold  Threshold=0.5  SaturateOnIntegerOverflow=off  InputSameDT=off
  sel : Constant  Value=double(sel_type == 1)
  y : Outport
  wires:
  a/1 -> Switch/1
  sel/1 -> Switch/2
  b/1 -> Switch/3
  Switch/1 -> y/1

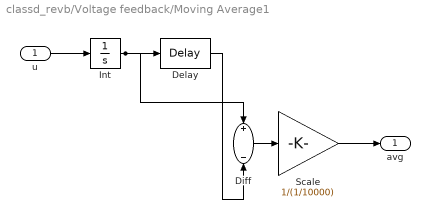
== system classd_revb/Voltage feedback/Moving Average1 ==
  u : Inport
  Delay : TransportDelay  DelayTime=1/10000  BufferSize=131072
  Diff : Sum  Inputs=+-
  Int : Integrator
  Scale : Gain  Gain=1/(1/10000)
  avg : Outport
  wires:
  Scale/1 -> avg/1
  u/1 -> Int/1
  Int/1 -> Diff/1, Delay/1
  Delay/1 -> Diff/2
  Diff/1 -> Scale/1

== system classd_revb/Demand/Sine Sweep/Ramp ==
  Limit : Saturate  UpperLimit=max(sweep_fStart,sweep_fEnd)  LowerLimit=min(sweep_fStart,sweep_fEnd)
  Ramp : Fcn  Expr=(sweep_fStart) + ((sweep_fEnd - sweep_fStart)/Timespan)*(u(1)-(0))*(u(1)>(0))
  t : Clock
  y : Outport
  wires:
  t/1 -> Ramp/1
  Ramp/1 -> Limit/1
  Limit/1 -> y/1

== matlab function classd_revb/Power stage (ideal switches)/classd_plant ==
  data: dx output; x input; y output; g input; ipos input; eload input; Pcd parameter
function [dx, y] = classd_plant(x, g, ipos, eload, Pcd)
%CLASSD_PLANT  Ideal-switch power stage of "Class D Rev B.plecs" (body of a MATLAB Function block).
%
% Six half bridges ("Half Bridge A".."F") on one DC bus. A, B, C drive the positive output
% node P through the leg inductors, D, E, F drive the negative node N. The load sits between
% P and N (Aout / Vout). The DC bus is the 18 mF bank (with ESR, plus the half-bridge local
% 10 uF capacitors lumped in) fed by the "AC_DC" block: a 100 A current source clamped by a
% 400 V zener and a series diode, i.e. a 400 V supply with a 100 A current limit.
%
% IGBTs/diodes are ideal: a leg with both gates off (dead time) is clamped by the diode chosen
% by the sign of its current. The IGBT/diode forward drops, snubbers, 82 nF film capacitors
% and the thermal network are not modelled.
%
% States  x = [iA; iB; iC; iD; iE; iF; vCB; vRC]
%   iA..iF  leg currents, positive flowing out of the leg midpoint ("Am1" in each half bridge)
%   vCB     DC bank capacitor voltage (behind its ESR)
%   vRC     voltage of the optional parallel R||C section of the load
% Inputs
%   g      12 gates [A_top A_bot B_top B_bot ... F_top F_bot]
%   ipos   6 booleans, leg current > 0 (zero-crossing events for the diodes)
%   eload  voltage of the optional source in series with the load (V)
% Outputs
%   y = [Vout; Iout; Vbus; Isupply; iA; iB; iC; iD; iE; iF; vP; vN]
%#codegen

P = Pcd;   % parameter struct from the workspace

il = x(1:6);
vCB = x(7);
vRC = x(8);
gd = double(g);
pd = double(ipos);

u = zeros(6, 1);
for k = 1:6
    top = gd(2*k - 1);
    bot = gd(2*k);
    if top > 0.5
        u(k) = 1;
    elseif bot > 0.5
        u(k) = 0;
    elseif pd(k) > 0.5          % current out of the midpoint -> bottom diode conducts
        u(k) = 0;
    else
        u(k) = 1;
    end
end

% --- DC bus: bank (vCB behind Resr) + current-limited supply --------------------------------
ibr = sum(u .* il);                        % current drawn from DC+ by the six legs
v1 = vCB + P.Resr * (P.Idc - ibr);         % bus voltage if the supply delivers its full Idc
if v1 <= P.Vz
    isup = P.Idc;
    vbus = v1;
else
    % zener conducting: isup = Idc - (vbus - Vz)/Rz
    vbus = (vCB + P.Resr * (P.Idc + P.Vz / P.Rz - ibr)) / (1 + P.Resr / P.Rz);
    isup = P.Idc - (vbus - P.Vz) / P.Rz;
    if isup < 0                              % series diode blocks reverse current
        isup = 0;
        vbus = vCB - P.Resr * ibr;
    end
end

% --- AC side: leg inductors into nodes P / N, load between P and N --------------------------
e = u * vbus - P.Rleg .* il;               % leg EMF behind each inductor
a = 1 ./ P.Lleg;
AP = sum(a(1:3));
AN = sum(a(4:6));
SP = sum(a(1:3) .* e(1:3));
SN = sum(a(4:6) .* e(4:6));
iL = sum(il(1:3));                         % load current (P -> N)
if P.has_rc > 0.5
    vrc = vRC;
else
    vrc = 0;
end
V0 = P.Rload * iL + vrc + P.E_on * eload;
diL = (SP / AP - SN / AN - V0) / (P.Lload + 1 / AP + 1 / AN);
vP = (SP - diL) / AP;
vN = (SN + diL) / AN;

dx = zeros(8, 1);
dx(1:3) = a(1:3) .* (e(1:3) - vP);
dx(4:6) = a(4:6) .* (e(4:6) - vN);
dx(7) = (isup - ibr) / P.CB;
if P.has_rc > 0.5
    dx(8) = (iL - vRC / P.Rpar) / P.Cpar;
end

y = [vP - vN; iL; vbus; isup; il; vP; vN];
end
